simulink model "swingup_lyapunov"  (R2024b)
settings: Solver=ode1  StartTime=0.0  StopTime=inf  FixedStep=0.002  RelTol=1e-3  EnableMultiTasking=on
settings Model: ExtModeTrigDuration=10000  Creator=nsoldati  LastModifiedBy=nikschmid
settings SolverCC: AlgebraicLoopSolver=TrustRegion  PositivePriorityOrder=on
settings DataIOCC: ReturnWorkspaceOutputs=off
settings OptimizationCC: ReuseModelBlockBuffer=off
settings DebuggingCC: UnconnectedInputMsg=warning  UnconnectedOutputMsg=warning  UnconnectedLineMsg=warning  ArithmeticOperatorsInVariantConditions=warning
settings ModelReferenceCC: EnableRefExpFcnMdlSchedulingChecks=on
settings SFSimCC: SimUseLocalCustomCode=off  CustomCodeUndefinedFunction=UseInterfaceOnly
settings RTWCC: Description=QUARC Win64 Target Using Toolchain  SystemTargetFile=quarc_win64.tlc  TemplateMakefile=quarc_default_tmf  RTWUseLocalCustomCode=off  Toolchain=QUARC win64 | nmake (64-bit Windows)  BuildConfiguration=Faster Runs  GPUComputeCapability=3.5
settings CodeAppCC: StateflowObjectComments=on
settings STFCustomTargetCC: TargetLangStandard=C99 (ISO)  ConcurrentExecutionCompliant=on  GRTInterface=on  UseToolchainInfoCompliant=on  SystemTargetFile=quarc_win64.tlc
settings GRTTargetCC: ParMdlRefBuildCompliant=off  CompOptLevelCompliant=off  CombineOutputUpdateFcns=off  MatFileLogging=off  CPPClassGenCompliant=off  GRTInterface=on  ExtMode=on  ExtModeMexFile=quarc_comm
settings ConfigComp: CovMetricSettings=dswe

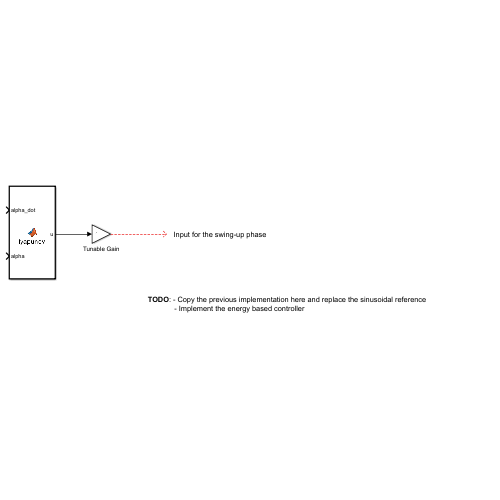
[thumbnail: Simulink's stored preview of the top-level diagram]
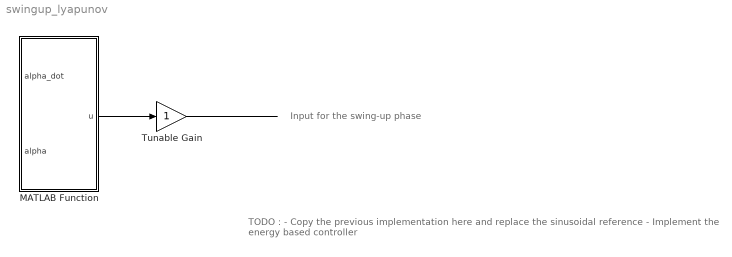
== system swingup_lyapunov ==
  note: Input for the swing-up phase
  note: TODO : - Copy the previous implementation here and replace the sinusoidal reference
      | - Implement the energy based controller
  MATLAB Function : MATLAB Function  TreatAsAtomicUnit=on
  Tunable Gain : Gain
  wires:
  MATLAB Function/1(u) -> Tunable Gain/1
  Tunable Gain/1 -> ?

== matlab function swingup_lyapunov/MATLAB Function ==
  data: alpha_dot input; u output; alpha input
% Following the theory of the script, find the optimal input signal given
% the values of the angle and the angular position.

% HINT: In the "active" regions, set |u| = 1, and adjust the amplitude with
% the simulink gain block (allows online tuning)

function u = lyapunov(alpha_dot, alpha)
    
end
